simulink model "mass_system_kalman"  (R2025a)
settings: Solver=VariableStepAuto  StartTime=0.0  StopTime=10.0  MaxStep=1e-3  RelTol=1e-3
values from neighbouring files (symbols this model uses):
  A = [0 1; -k/m -c/m]    [kalman_filter_spring.m]
  B = [0 1/m]'    [kalman_filter_spring.m]
  C = eye(2)    [kalman_filter_spring.m]
  c_delta = c  * 0.95    (= 0.57)    [kalman_filter_spring.m]
  D = zeros(2, 1)    [kalman_filter_spring.m]
  F = [1 - k/(2*m)*Ts^2, Ts - c/(2*m)*Ts^2 ... (first row only)    [kalman_filter_spring.m]
  G = [1/(2*m)*Ts^2 ... (first row only)    [kalman_filter_spring.m]
  Gs = ss(A, B, C, D)    [kalman_filter_spring.m]
  H = eye(2)    [kalman_filter_spring.m]
  R = diag([sigma_p1^2 , sigma_v1^2])    [kalman_filter_spring.m]
  Ts = 1/Fs    (= 0.001)    [kalman_filter_spring.m]
undefined symbols (not defined in the file or in its folder): Discrete, Time
libraries: fl_lib x6, nesl_utility x4, ctrlSharedLib x1, simulink x1, sdl_lib x1
settings Model: Creator=amoralesma  LastModifiedBy=amoralesma

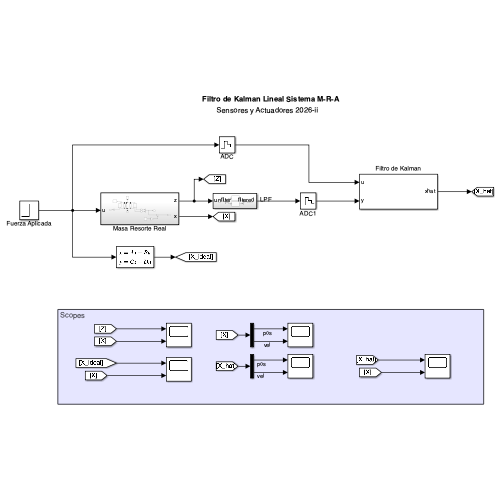
[thumbnail: Simulink's stored preview of the top-level diagram]
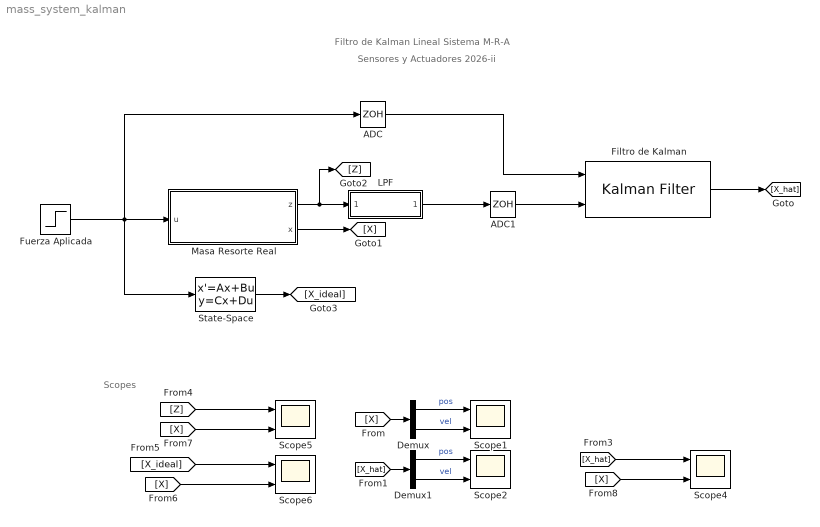
== system mass_system_kalman ==
  note: Filtro de Kalman Lineal Sistema M-R-A
  note: Scopes
  note: Sensores y Actuadores 2026-ii
  ADC : ZeroOrderHold  SampleTime=Ts
  ADC1 : ZeroOrderHold  SampleTime=Ts
  Demux : Demux  Outputs=2
  Demux1 : Demux  Outputs=2
  Filtro de Kalman : ctrlSharedLib/Kalman Filter  TimeDomain=Discrete-Time  UseCurrentEstimator=on  ModelSource=Individual A, B, C, D matrices  ModelSourceVariable=c2d(Gs, 1/100, 'zoh');  A=F  B=G  C=H  D=D  NumberOfStates=1  NumberOfInputs=1  NumberOfOutputs=1  InitialEstimateSource=Dialog  X0=[0 0]  P0=10  UseK=off  UseGH=off  NumberOfProcessNoiseInputs=1  G=1  TimeInvariantG=on  H=0  TimeInvariantH=on  Q=Q  TimeInvariantQ=on  R=R  TimeInvariantR=on  N=0  TimeInvariantN=on  AddInputPort=on  AddEnablePort=off  OutputEstimatedY=off  OutputP=off  Ts=Ts
  Fuerza Aplicada : Step  After=10  SampleTime=0
  LPF : Subsystem
  Masa Resorte Real : Subsystem
  Scope{1..2,4..6} (5 alike) : Scope  NumInputPorts=2
      Scope1 settings: ActiveDisplayYMinimum=-0.2573798131888474  ActiveDisplayYMaximum=2.3164183186996272
      Scope2 settings: ActiveDisplayYMinimum=-2.6231814437104823  ActiveDisplayYMaximum=7.7529024239317472
      Scope4 settings: ActiveDisplayYMinimum=0.7595735549500342  ActiveDisplayYMaximum=2.6805074594725204  DataLoggingVariableName=ScopeData3
      Scope5 settings: ActiveDisplayYMinimum=-3.5871974554150308  ActiveDisplayYMaximum=9.5913024287549682  DataLoggingVariableName=ScopeData4
      Scope6 settings: ActiveDisplayYMinimum=-0.82407539964366716  ActiveDisplayYMaximum=5.6704745865453283  DataLoggingVariableName=ScopeData5
  State-Space : StateSpace  A=A  B=B  C=C  D=zeros(2,1)  InitialCondition=0
  wires:
  Fuerza Aplicada/1 -> State-Space/1, Masa Resorte Real/1(u), ADC/1
  [X] -> Demux/1
  Demux/1 -> Scope1/1  "pos"
  Demux/2 -> Scope1/2  "vel"
  ADC/1 -> Filtro de Kalman/1
  Filtro de Kalman/1 -> [X_hat]
  [X_hat] -> Demux1/1
  Demux1/1 -> Scope2/1  "pos"
  Demux1/2 -> Scope2/2  "vel"
  Masa Resorte Real/2(x) -> [X]
  ADC1/1 -> Filtro de Kalman/2
  [Z] -> Scope5/1
  Masa Resorte Real/1(z) -> LPF/1(unfilter), [Z]
  State-Space/1 -> [X_ideal]
  [X_ideal] -> Scope6/1
  [X] -> Scope6/2
  [X] -> Scope5/2
  LPF/1(filtered) -> ADC1/1
  [X_hat] -> Scope4/1
  [X] -> Scope4/2

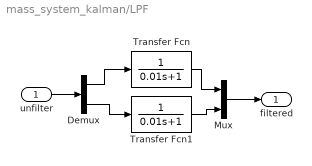
== system mass_system_kalman/LPF ==
  unfilter : Inport
  Demux : Demux  Outputs=2
  Mux : Mux  Inputs=2
  Transfer Fcn : TransferFcn  Denominator=[0.01 1]
  Transfer Fcn1 : TransferFcn  Denominator=[0.01 1]
  filtered : Outport
  wires:
  unfilter/1 -> Demux/1
  Demux/1 -> Transfer Fcn/1
  Demux/2 -> Transfer Fcn1/1
  Transfer Fcn/1 -> Mux/1
  Transfer Fcn1/1 -> Mux/2
  Mux/1 -> filtered/1

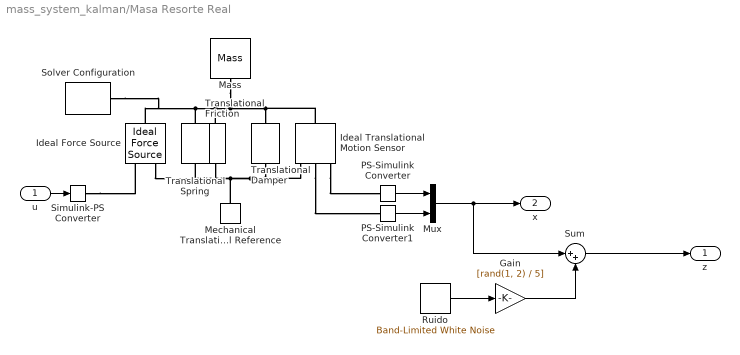
== system mass_system_kalman/Masa Resorte Real ==
  u : Inport
  Gain : Gain  Gain=[rand(1, 2) / 5]
  Ideal Force Source : fl_lib/Mechanical/Mechanical Sources/Ideal Force Source
  Ideal Translational Motion Sensor : fl_lib/Mechanical/Mechanical Sensors/Ideal Translational Motion Sensor  reference=foundation.enum.MeasurementReference.difference  acceleration_port=false  velocity_port=true  position_port=true  offset=0 m
  Mass : fl_lib/Mechanical/Translational Elements/Mass  mass=m_delta kg  num_ports=foundation.enum.numPorts2.one  v_specify=off  v_priority=High  v=0 m/s  v_nominal_specify=off  v_nominal_value=1  v_nominal_unit=m/s  f_specify=off  f_priority=None  f=0 N  f_nominal_specify=off  f_nominal_value=1  f_nominal_unit=N
  Mechanical Translational Reference : fl_lib/Mechanical/Translational Elements/Mechanical Translational Reference
  Mux : Mux  Inputs=2
  PS-Simulink Converter : nesl_utility/PS-Simulink Converter  PhysicalDomain=network_engine_domain  SubClassName=ps_output  LeftPortType=input  RightPortType=output  PseudoPeriodic=off  Frequencies=[]  VectorFormat=inherit  Unit=inherit  AffineConversion=off
  PS-Simulink Converter1 : nesl_utility/PS-Simulink Converter  PhysicalDomain=network_engine_domain  SubClassName=ps_output  LeftPortType=input  RightPortType=output  PseudoPeriodic=off  Frequencies=[]  VectorFormat=inherit  Unit=inherit  AffineConversion=off
  Ruido : simulink/Sources/Band-Limited White Noise  Cov=[0.001]  Ts=1e-3  seed=[23341]
  Simulink-PS Converter : nesl_utility/Simulink-PS Converter  PhysicalDomain=network_engine_domain  SubClassName=ps_input  LeftPortType=input  RightPortType=output  PseudoPeriodic=off  Frequencies=[]  NoiseDistribution=none  NoiseParameters=[]  Unit=1  AffineConversion=off  FilteringAndDerivatives=provide  SimscapeFilterOrder=1  InputFilterTimeConstant=0.001  UdotUserProvided=0
  Solver Configuration : nesl_utility/Solver Configuration  PhysicalDomain=network_engine_domain  SubClassName=solver  LeftPortType=input  RightPortType=generic  Tones=[]  Harmonics=[]  SimulateNoise=off  Profile=off  UseLocalSampling=off  EnableSwitchedLinearOptims=on  FrequencyDomain=off  UseCCode=off  RelTol=0.001  AbsTol=0.001  MinStep=1e-09  ToWorkspace=off  RevertToSquareIcSolve=off  NumHomotopyIterations=100  PhasorMode=off  PhasorModeNumHarmonics=1  ConsistencySolver=NEWTON_XTOL_AFTER_FTOL  IndexReductionMethod=DerivativeReplacement  DoDC=off  ResidualTolerance=1e-09  ConsistencyTolSource=GLOBAL  ConsistencyAbsTol=0.001  ConsistencyRelTol=0.001  ConsistencyTolFactor=0.001  UseLocalSolver=off  LocalSolverChoice=NE_BACKWARD_EULER_ADVANCER  ResolveIndetEquations=on  FunctionEvalNumThread=1  LocalSolverSampleTime=0.001  DoFixedCost=off  MaxNonlinIter=3  MaxModeIter=2  ComputeImpulses=off  ImpulseIterations=2  LinearAlgebra=auto  LinearAlgebraNumThread=0  EquationFormulation=NE_TIME_EF  DelaysMemoryBudget=1024  AutomaticFiltering=on  FilteringTimeConstant=0.001  PartitionStorageMethod=AS_NEEDED  PartitionMemoryBudget=1024  PartitionMethod=ROBUST  MultibodyUseLocalSolver=off  MultibodyLocalSolverChoice=ODE1  MultibodyLocalSolverSampleTime=0.001
  Sum : Sum  Inputs=|++
  Translational Friction : fl_lib/Mechanical/Translational Elements/Translational Friction  brkwy_frc=1.1 N  brkwy_vel=1.1 m/s  Col_frc=1 N  visc_coef=1e-1 N*s/m  v_specify=off  v_priority=None  v=0 m/s  v_nominal_specify=off  v_nominal_value=1  v_nominal_unit=m/s  f_specify=off  f_priority=None  f=0 N  f_nominal_specify=off  f_nominal_value=1  f_nominal_unit=N
      settings: InternalSimscapePortConfiguration="{\"Bottom\":[],\"Left\":[{\"id\":\"R\",\"label\":\"R\",\"type\":\"foundation.mechanical.translational.translational\"}],\"Right\":[{\"id\":\"C\",\"label\":\"C\",\"type\":\"foundation.mechanical.translational.translational\"}],\"Top\":[]}"
  Translational Damper : sdl_lib/Couplings & Drives/Springs & Dampers/Translational Damper  D=c_delta N*s/m  thermal_port=simscape.enum.thermaleffects.omit  thermal_mass=50 kJ/K  temperature_specify=off  temperature_priority=High  temperature=300 K  temperature_nominal_specify=off  temperature_nominal_value=1  temperature_nominal_unit=K
  Translational Spring : fl_lib/Mechanical/Translational Elements/Translational Spring  spr_rate=k_delta N/m  v_specify=off  v_priority=None  v=0 m/s  v_nominal_specify=off  v_nominal_value=1  v_nominal_unit=m/s  f_specify=off  f_priority=None  f=0 N  f_nominal_specify=off  f_nominal_value=1  f_nominal_unit=N  x_specify=off  x_priority=High  x=0 m  x_nominal_specify=off  x_nominal_value=1  x_nominal_unit=m
  z : Outport
  x : Outport  Port=2
  wires:
  Mux/1 -> Sum/1, x/1
  PS-Simulink Converter/1 -> Mux/1
  u/1 -> Simulink-PS Converter/1
  PS-Simulink Converter1/1 -> Mux/2
  Ruido/1 -> Gain/1
  Gain/1 -> Sum/2
  Sum/1 -> z/1
  connections:
  Ideal Translational Motion Sensor/RConn2 -- PS-Simulink Converter1/LConn1
  Simulink-PS Converter/RConn1 -- Ideal Force Source/RConn1
  Ideal Translational Motion Sensor/RConn3 -- PS-Simulink Converter/LConn1
  Translational Spring/LConn1 -- Translational Friction/LConn1 -- Ideal Translational Motion Sensor/LConn1 -- Translational Damper/LConn1 -- Mass/LConn1 -- Solver Configuration/RConn1 -- Ideal Force Source/LConn1
  Translational Damper/RConn1 -- Translational Friction/RConn1 -- Ideal Force Source/RConn2 -- Translational Spring/RConn1 -- Mechanical Translational Reference/LConn1 -- Ideal Translational Motion Sensor/RConn1
